simulink model "AXU5EV_Experiment_Control_Angle_HDL"  (R2026b)
settings: Solver=FixedStepDiscrete  StopTime=2  FixedStep=1
settings Model: Creator=lww  LastModifiedBy=lww

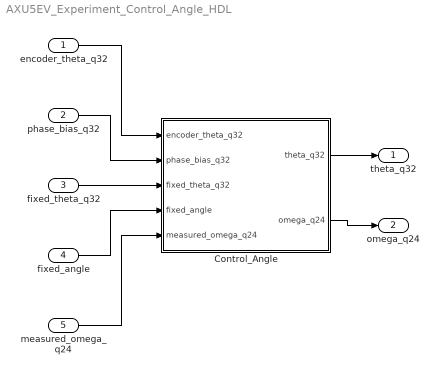
== system AXU5EV_Experiment_Control_Angle_HDL ==
  encoder_theta_q32 : Inport  OutDataTypeStr=int64
  phase_bias_q32 : Inport  Port=2  OutDataTypeStr=int64
  fixed_theta_q32 : Inport  Port=3  OutDataTypeStr=int64
  fixed_angle : Inport  Port=4  OutDataTypeStr=boolean
  measured_omega_q24 : Inport  Port=5  OutDataTypeStr=int64
  Control_Angle : Subsystem
  theta_q32 : Outport
  omega_q24 : Outport  Port=2
  wires:
  Control_Angle/2(omega_q24) -> omega_q24/1
  Control_Angle/1(theta_q32) -> theta_q32/1
  measured_omega_q24/1 -> Control_Angle/5(measured_omega_q24)
  fixed_angle/1 -> Control_Angle/4(fixed_angle)
  fixed_theta_q32/1 -> Control_Angle/3(fixed_theta_q32)
  phase_bias_q32/1 -> Control_Angle/2(phase_bias_q32)
  encoder_theta_q32/1 -> Control_Angle/1(encoder_theta_q32)

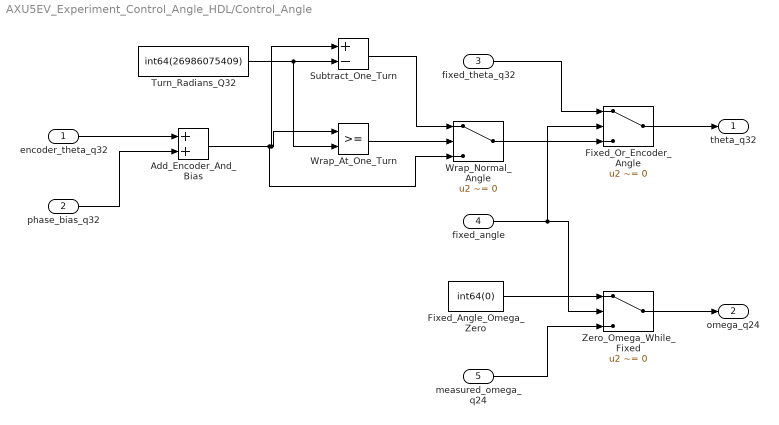
== system AXU5EV_Experiment_Control_Angle_HDL/Control_Angle ==
  encoder_theta_q32 : Inport
  phase_bias_q32 : Inport  Port=2
  fixed_theta_q32 : Inport  Port=3
  fixed_angle : Inport  Port=4
  measured_omega_q24 : Inport  Port=5
  Add_Encoder_And_Bias : Sum  OutDataTypeStr=int64
  Fixed_Angle_Omega_Zero : Constant  Value=int64(0)  OutDataTypeStr=int64
  Fixed_Or_Encoder_Angle : Switch  Criteria=u2 ~= 0  SaturateOnIntegerOverflow=off  InputSameDT=off
  Subtract_One_Turn : Sum  Inputs=+-  OutDataTypeStr=int64
  Turn_Radians_Q32 : Constant  Value=int64(26986075409)  OutDataTypeStr=int64
  Wrap_At_One_Turn : RelationalOperator  OutDataTypeStr=boolean  RndMeth=Simplest  InputSameDT=off
  Wrap_Normal_Angle : Switch  Criteria=u2 ~= 0  SaturateOnIntegerOverflow=off  InputSameDT=off
  Zero_Omega_While_Fixed : Switch  Criteria=u2 ~= 0  SaturateOnIntegerOverflow=off  InputSameDT=off
  theta_q32 : Outport
  omega_q24 : Outport  Port=2
  wires:
  Zero_Omega_While_Fixed/1 -> omega_q24/1
  measured_omega_q24/1 -> Zero_Omega_While_Fixed/3
  Fixed_Angle_Omega_Zero/1 -> Zero_Omega_While_Fixed/1
  Fixed_Or_Encoder_Angle/1 -> theta_q32/1
  Wrap_Normal_Angle/1 -> Fixed_Or_Encoder_Angle/3
  fixed_angle/1 -> Fixed_Or_Encoder_Angle/2, Zero_Omega_While_Fixed/2
  fixed_theta_q32/1 -> Fixed_Or_Encoder_Angle/1
  Wrap_At_One_Turn/1 -> Wrap_Normal_Angle/2
  Subtract_One_Turn/1 -> Wrap_Normal_Angle/1
  Turn_Radians_Q32/1 -> Subtract_One_Turn/2, Wrap_At_One_Turn/2
  Add_Encoder_And_Bias/1 -> Subtract_One_Turn/1, Wrap_At_One_Turn/1, Wrap_Normal_Angle/3
  phase_bias_q32/1 -> Add_Encoder_And_Bias/2
  encoder_theta_q32/1 -> Add_Encoder_And_Bias/1
